simulink model "SteeringColumn_s"  (R2023a)
settings: Solver=VariableStepAuto  StartTime=0.0  StopTime=10.0  RelTol=1e-3
undefined symbols (not defined in the file): c, C1, C2, J1, J2, K, T_f
settings Model: Creator=Tan_Tram  LastModifiedBy=Tan_Tram

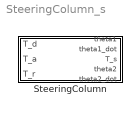
== system SteeringColumn_s ==
  SteeringColumn : Subsystem

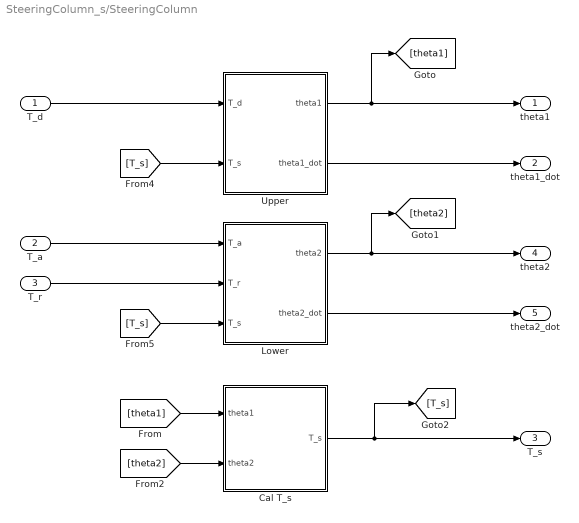
== system SteeringColumn_s/SteeringColumn ==
  T_d : Inport
  T_a : Inport  Port=2
  T_r : Inport  Port=3
  Cal T_s : Subsystem
  Lower : Subsystem
  Upper : Subsystem
  theta1 : Outport
  theta1_dot : Outport  Port=2
  T_s : Outport  Port=3
  theta2 : Outport  Port=4
  theta2_dot : Outport  Port=5
  wires:
  T_d/1 -> Upper/1(T_d)
  T_a/1 -> Lower/1(T_a)
  T_r/1 -> Lower/2(T_r)
  [theta1] -> Cal T_s/1(theta1)
  Upper/1(theta1) -> theta1/1, [theta1]
  [theta2] -> Cal T_s/2(theta2)
  Lower/1(theta2) -> theta2/1, [theta2]
  [T_s] -> Upper/2(T_s)
  [T_s] -> Lower/3(T_s)
  Cal T_s/1(T_s) -> T_s/1, [T_s]
  Upper/2(theta1_dot) -> theta1_dot/1
  Lower/2(theta2_dot) -> theta2_dot/1

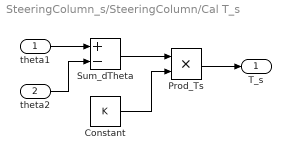
== system SteeringColumn_s/SteeringColumn/Cal T_s ==
  theta1 : Inport
  theta2 : Inport  Port=2
  Constant : Constant  Value=K
  Prod_Ts : Product  Inputs=**
  Sum_dTheta : Sum  Inputs=+-
  T_s : Outport
  wires:
  Constant/1 -> Prod_Ts/2
  Sum_dTheta/1 -> Prod_Ts/1
  theta1/1 -> Sum_dTheta/1
  Prod_Ts/1 -> T_s/1
  theta2/1 -> Sum_dTheta/2

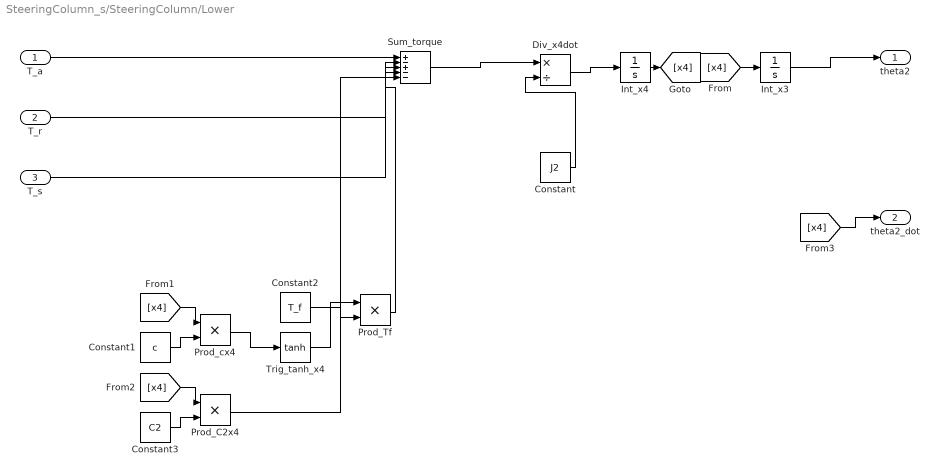
== system SteeringColumn_s/SteeringColumn/Lower ==
  T_a : Inport
  T_r : Inport  Port=2
  T_s : Inport  Port=3
  Constant : Constant  Value=J2
  Constant1 : Constant  Value=c
  Constant2 : Constant  Value=T_f
  Constant3 : Constant  Value=C2
  Div_x4dot : Product  Inputs=*/
  Int_x3 : Integrator
  Int_x4 : Integrator
  Prod_C2x4 : Product  Inputs=**
  Prod_Tf : Product  Inputs=**
  Prod_cx4 : Product  Inputs=**
  Sum_torque : Sum  Inputs=+-+--
  Trig_tanh_x4 : Trigonometry  Operator=tanh
  theta2 : Outport
  theta2_dot : Outport  Port=2
  wires:
  Int_x4/1 -> [x4]
  [x4] -> Prod_cx4/1
  Constant1/1 -> Prod_cx4/2
  Prod_cx4/1 -> Trig_tanh_x4/1
  Trig_tanh_x4/1 -> Prod_Tf/1
  Constant2/1 -> Prod_Tf/2
  [x4] -> Prod_C2x4/1
  Constant3/1 -> Prod_C2x4/2
  T_a/1 -> Sum_torque/1
  T_r/1 -> Sum_torque/2
  T_s/1 -> Sum_torque/3
  Prod_Tf/1 -> Sum_torque/4
  Prod_C2x4/1 -> Sum_torque/5
  Sum_torque/1 -> Div_x4dot/1
  Constant/1 -> Div_x4dot/2
  Div_x4dot/1 -> Int_x4/1
  [x4] -> Int_x3/1
  Int_x3/1 -> theta2/1
  [x4] -> theta2_dot/1

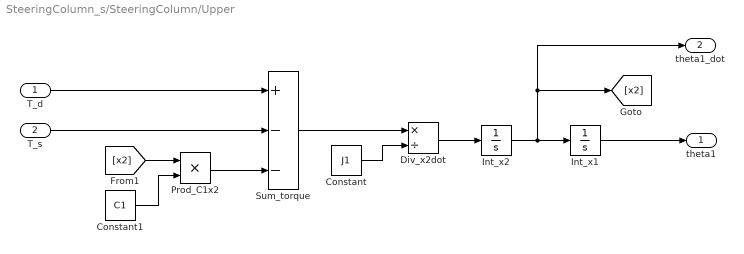
== system SteeringColumn_s/SteeringColumn/Upper ==
  T_d : Inport
  T_s : Inport  Port=2
  Constant : Constant  Value=J1
  Constant1 : Constant  Value=C1
  Div_x2dot : Product  Inputs=*/
  Int_x1 : Integrator
  Int_x2 : Integrator
  Prod_C1x2 : Product  Inputs=**
  Sum_torque : Sum  Inputs=+--
  theta1 : Outport
  theta1_dot : Outport  Port=2
  wires:
  T_d/1 -> Sum_torque/1
  Sum_torque/1 -> Div_x2dot/1
  Constant1/1 -> Prod_C1x2/2
  Int_x2/1 -> Int_x1/1, theta1_dot/1, [x2]
  Prod_C1x2/1 -> Sum_torque/3
  Int_x1/1 -> theta1/1
  [x2] -> Prod_C1x2/1
  T_s/1 -> Sum_torque/2
  Constant/1 -> Div_x2dot/2
  Div_x2dot/1 -> Int_x2/1
